simulink model "BMS_OC_Protection_Test"  (R2025b)
settings: Solver=FixedStepDiscrete  StartTime=0.0  StopTime=1  FixedStep=Ts  RelTol=1e-3
undefined symbols (not defined in the file): Ts
settings Model: Creator=Khadija  LastModifiedBy=Khadija

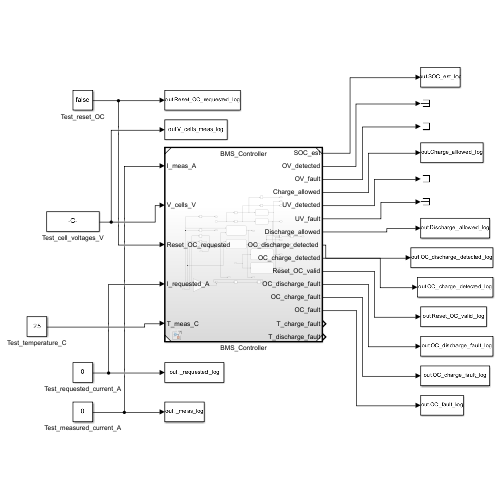
[thumbnail: Simulink's stored preview of the top-level diagram]
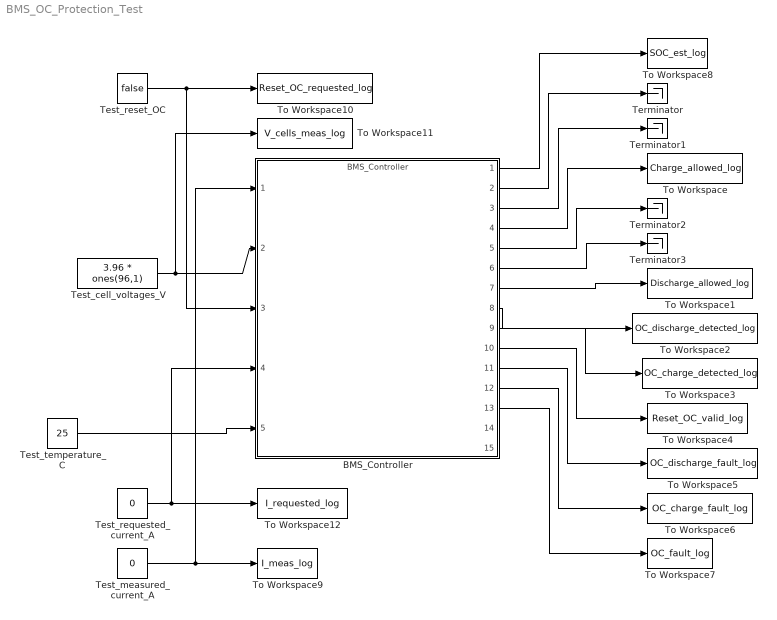
== system BMS_OC_Protection_Test ==
  BMS_Controller : ModelReference  ModelNameDialog=BMS_Controller.slx  SimulationMode=Normal  ModelReferenceVersion=1.40
  Terminator{,1..3} (4 alike) : Terminator
  Test_cell_voltages_V : Constant  Value=3.96 * ones(96,1)  SampleTime=Ts
  Test_measured_current_A : Constant  Value=0  SampleTime=Ts
  Test_requested_current_A : Constant  Value=0  SampleTime=Ts
  Test_reset_OC : Constant  Value=false  SampleTime=Ts
  Test_temperature_C : Constant  Value=25  OutDataTypeStr=double  SampleTime=Ts
  To Workspace : ToWorkspace  VariableName=Charge_allowed_log  SaveFormat=Timeseries  SampleTime=-1
  To Workspace1 : ToWorkspace  VariableName=Discharge_allowed_log  SaveFormat=Timeseries  SampleTime=-1
  To Workspace10 : ToWorkspace  VariableName=Reset_OC_requested_log  SaveFormat=Timeseries  SampleTime=-1
  To Workspace11 : ToWorkspace  VariableName=V_cells_meas_log  SaveFormat=Timeseries  SampleTime=-1
  To Workspace12 : ToWorkspace  VariableName=I_requested_log  SaveFormat=Timeseries  SampleTime=-1
  To Workspace2 : ToWorkspace  VariableName=OC_discharge_detected_log  SaveFormat=Timeseries  SampleTime=-1
  To Workspace3 : ToWorkspace  VariableName=OC_charge_detected_log  SaveFormat=Timeseries  SampleTime=-1
  To Workspace4 : ToWorkspace  VariableName=Reset_OC_valid_log  SaveFormat=Timeseries  SampleTime=-1
  To Workspace5 : ToWorkspace  VariableName=OC_discharge_fault_log  SaveFormat=Timeseries  SampleTime=-1
  To Workspace6 : ToWorkspace  VariableName=OC_charge_fault_log  SaveFormat=Timeseries  SampleTime=-1
  To Workspace7 : ToWorkspace  VariableName=OC_fault_log  SaveFormat=Timeseries  SampleTime=-1
  To Workspace8 : ToWorkspace  VariableName=SOC_est_log  SaveFormat=Timeseries  SampleTime=-1
  To Workspace9 : ToWorkspace  VariableName=I_meas_log  SaveFormat=Timeseries  SampleTime=-1
  wires:
  Test_reset_OC/1 -> BMS_Controller/3, To Workspace10/1
  Test_requested_current_A/1 -> To Workspace12/1, BMS_Controller/4
  Test_cell_voltages_V/1 -> To Workspace11/1, BMS_Controller/2
  Test_measured_current_A/1 -> BMS_Controller/1, To Workspace9/1
  BMS_Controller/1 -> To Workspace8/1
  BMS_Controller/2 -> Terminator/1
  BMS_Controller/3 -> Terminator1/1
  BMS_Controller/7 -> To Workspace1/1
  BMS_Controller/6 -> Terminator3/1
  BMS_Controller/5 -> Terminator2/1
  BMS_Controller/4 -> To Workspace/1
  BMS_Controller/11 -> To Workspace5/1
  BMS_Controller/10 -> To Workspace4/1
  BMS_Controller/9 -> To Workspace3/1
  BMS_Controller/8 -> To Workspace2/1
  BMS_Controller/13 -> To Workspace7/1
  BMS_Controller/12 -> To Workspace6/1
  Test_temperature_C/1 -> BMS_Controller/5
